simulink model "wing_example_unst_sim"  (R2018b)
settings: Solver=VariableStepAuto  StartTime=0.0  StopTime=1000.0  FixedStep=0.0001  RelTol=1e-3
values from neighbouring files (symbols this model uses):
  wing = wingSetState(wing, alpha, beta, V, omega,      actuators_pos, actuators_rate, xyz_cg, 'atmosphere', isAtmosphere(h),      'V_Wb', zeros( 3, wing.n_panel ), 'V_Wb_dt', zeros( 3, wing.n_panel ) )    [wing_example.m]    (also in wing_example_Arkbird.m = wingSetState(wing, alpha, beta, V, omega,      actuators_pos; wing_example_geometry_from_CPACS.m = wingSetState(wing, alpha, beta, V, omega,      [ actuatorsLe; wing_example_polar.m = wingCreate('wing_params_Arkbird_simple',50); wing_example_sim_init.m = wingCreate('wing_params_Arkbird_simple',30))
libraries: atmosphere_lib x1, vlm_wing_lib x1
settings Model: Creator=Yannic  LastModifiedBy=yannic

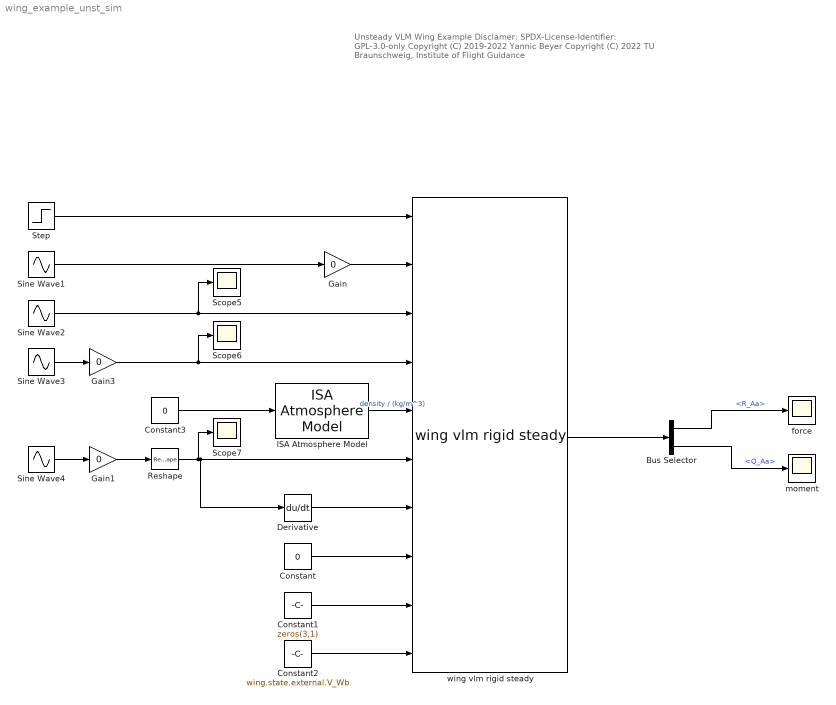
== system wing_example_unst_sim ==
  note: Unsteady VLM Wing Example
      |
      | Disclamer:
      | SPDX-License-Identifier: GPL-3.0-only
      |
      | Copyright (C) 2019-2022 Yannic Beyer
      | Copyright (C) 2022 TU Braunschweig, Institute of Flight Guidance
  Bus Selector : BusSelector  OutputSignals=R_Aa,Q_Aa
  Constant : Constant  Value=0
  Constant1 : Constant  Value=zeros(3,1)  VectorParams1D=off
  Constant2 : Constant  Value=wing.state.external.V_Wb
  Constant3 : Constant  Value=0
  Derivative : Derivative
  Gain : Gain  Gain=0
  Gain1 : Gain  Gain=0
  Gain3 : Gain  Gain=0
  ISA Atmosphere Model : atmosphere_lib/ISA Atmosphere Model
      settings: SourceProductName=LADAC
  Reshape : Reshape  OutputDimensionality=Row vector (2-D)
  Scope5 : Scope
  Scope6 : Scope
  Scope7 : Scope
  Sine Wave1 : Sin  Amplitude=0.05  Frequency=0.3  SampleTime=0
  Sine Wave2 : Sin  Amplitude=3  Bias=100  Frequency=0.22  SampleTime=0
  Sine Wave3 : Sin  Amplitude=[0.1;0.1;0.1]  Frequency=[0.9;0.8;0.7]  SampleTime=0
  Sine Wave4 : Sin  Amplitude=[0.1;0.1]  Frequency=[0.9;0.8]*2.1  SampleTime=0
  Step : Step  Time=0.01  After=0.1  SampleTime=0
  force : Scope
  moment : Scope
  wing vlm rigid steady : vlm_wing_lib/wing vlm rigid steady  wing_struct=wing  wing_state_bus=wing_state_bus  alpha_ind_init=0
      settings: SourceProductName=LADAC
  wires:
  Step/1 -> wing vlm rigid steady/1
  Sine Wave3/1 -> Gain3/1
  Sine Wave4/1 -> Gain1/1
  Reshape/1 -> Scope7/1, Derivative/1, wing vlm rigid steady/6
  Sine Wave1/1 -> Gain/1
  Gain/1 -> wing vlm rigid steady/2
  Gain1/1 -> Reshape/1
  Gain3/1 -> Scope6/1, wing vlm rigid steady/4
  Sine Wave2/1 -> Scope5/1, wing vlm rigid steady/3
  Constant/1 -> wing vlm rigid steady/8
  Constant1/1 -> wing vlm rigid steady/9
  wing vlm rigid steady/1 -> Bus Selector/1
  Bus Selector/1 -> force/1  "<R_Aa>"
  Bus Selector/2 -> moment/1  "<Q_Aa>"
  Constant2/1 -> wing vlm rigid steady/10
  ISA Atmosphere Model/1 -> wing vlm rigid steady/5  "density / (kg/m^3)"
  Constant3/1 -> ISA Atmosphere Model/1
  Derivative/1 -> wing vlm rigid steady/7
